simulink model "rate_channel"  (Simulink 4.00)
settings: Solver=ode45  StartTime=0.0  StopTime=100  RelTol=1e-3
libraries: simulink3 x2
settings Model: Creator=mcar  LastModifiedBy=mcar  BlockReductionOpt=off

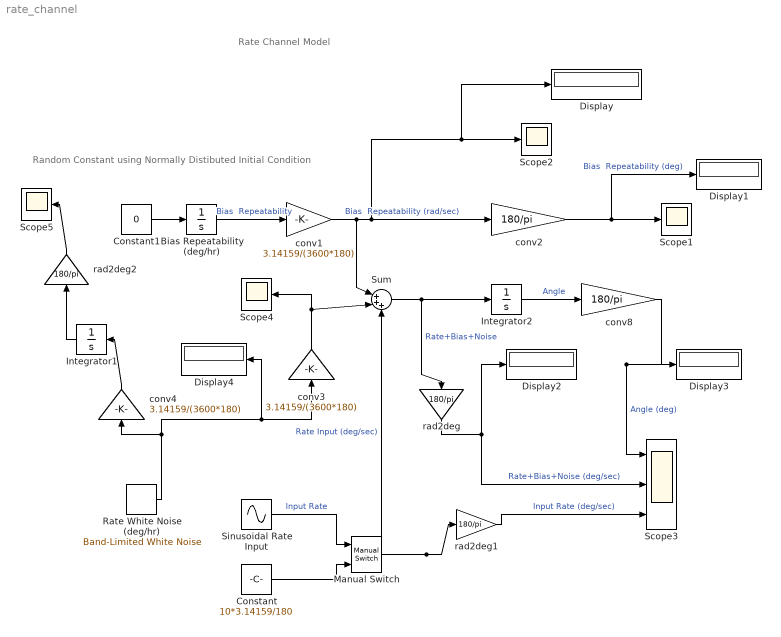
== system rate_channel ==
  note: Random Constant using
      | Normally Distibuted Initial Condition
  note: Rate Channel Model
  Bias Repeatability (deg/hr) : Integrator  ExternalReset=none  InitialConditionSource=internal  InitialCondition=10+3*rand  LimitOutput=off  UpperSaturationLimit=inf  LowerSaturationLimit=-inf  ShowSaturationPort=off  ShowStatePort=off  AbsoluteTolerance=auto
  Constant : Constant  Value=10*3.14159/180
  Constant1 : Constant  Value=0
  Display{,1..4} (5 alike) : Display
      settings: Format=short
  Integrator1 : Integrator  Orientation=left  ExternalReset=none  InitialConditionSource=internal  InitialCondition=0  LimitOutput=off  UpperSaturationLimit=inf  LowerSaturationLimit=-inf  ShowSaturationPort=off  ShowStatePort=off  AbsoluteTolerance=auto
  Integrator2 : Integrator  ExternalReset=none  InitialConditionSource=internal  InitialCondition=0  LimitOutput=off  UpperSaturationLimit=inf  LowerSaturationLimit=-inf  ShowSaturationPort=off  ShowStatePort=off  AbsoluteTolerance=auto
  Manual Switch : simulink3/Nonlinear/Manual Switch  sw=1  action=0
  Rate White Noise (deg/hr) : simulink3/Sources/Band-Limited White Noise  Cov=[360^2]  Ts=0.1  seed=[23341]
  Scope{1..2,4..5} (4 alike) : Scope
      Scope1 settings: TimeRange=auto  YMin=-5  YMax=5  SaveToWorkspace=off  SaveName=ScopeData  LimitDataPoints=on  MaxDataPoints=5000
      Scope2 settings: TimeRange=auto  YMin=-5  YMax=5  SaveToWorkspace=off  LimitDataPoints=on  MaxDataPoints=5000
      Scope4 settings: TimeRange=100  YMin=-0.02  YMax=0.03  SaveToWorkspace=off  SaveName=ScopeData3  LimitDataPoints=on  MaxDataPoints=5000
      Scope5 settings: TimeRange=auto  YMin=-5  YMax=5  SaveToWorkspace=off  SaveName=ScopeData4  LimitDataPoints=on  MaxDataPoints=5000
  Scope3 : Scope  NumInputPorts=3
      settings: TimeRange=auto  YMin=-0.1~-100~-100  YMax=0.8~100~100  SaveToWorkspace=off  SaveName=ScopeData2  LimitDataPoints=on  MaxDataPoints=5000
  Sinusoidal Rate Input : Sin  Amplitude=1  Frequency=10*pi/180/3600  Phase=0  SampleTime=0
  Sum : Sum  Inputs=|+++  SaturateOnIntegerOverflow=on
  conv1 : Gain  Gain=3.14159/(3600*180)  Multiplication=Element-wise(K.*u)  SaturateOnIntegerOverflow=on
  conv2 : Gain  Gain=180/pi  Multiplication=Element-wise(K.*u)  SaturateOnIntegerOverflow=on
  conv3 : Gain  Orientation=up  Gain=3.14159/(3600*180)  Multiplication=Element-wise(K.*u)  SaturateOnIntegerOverflow=on
  conv4 : Gain  Orientation=up  Gain=3.14159/(3600*180)  Multiplication=Element-wise(K.*u)  SaturateOnIntegerOverflow=on
  conv8 : Gain  Gain=180/pi  Multiplication=Element-wise(K.*u)  SaturateOnIntegerOverflow=on
  rad2deg : Gain  Orientation=down  Gain=180/pi  Multiplication=Element-wise(K.*u)  SaturateOnIntegerOverflow=on
  rad2deg1 : Gain  Gain=180/pi  Multiplication=Element-wise(K.*u)  SaturateOnIntegerOverflow=on
  rad2deg2 : Gain  Orientation=up  Gain=180/pi  Multiplication=Element-wise(K.*u)  SaturateOnIntegerOverflow=on
  wires:
  Bias Repeatability (deg/hr)/1 -> conv1/1  "Bias  Repeatability"
  Sum/1 -> Integrator2/1, rad2deg/1  "Rate+Bias+Noise"
  Rate White Noise (deg/hr)/1 -> conv3/1, Display4/1, conv4/1
  Integrator2/1 -> conv8/1  "Angle"
  conv8/1 -> Scope3/1, Display3/1  "Angle (deg)"
  conv1/1 -> Sum/1, conv2/1, Scope2/1, Display/1  "Bias  Repeatability (rad/sec)"
  conv2/1 -> Scope1/1, Display1/1  "Bias  Repeatability (deg)"
  conv3/1 -> Sum/2, Scope4/1
  rad2deg/1 -> Scope3/2, Display2/1  "Rate+Bias+Noise (deg/sec)"
  rad2deg1/1 -> Scope3/3  "Input Rate (deg/sec)"
  Constant/1 -> Manual Switch/2
  Sinusoidal Rate Input/1 -> Manual Switch/1  "Input Rate"
  Manual Switch/1 -> rad2deg1/1, Sum/3  "Rate Input (deg/sec)"
  Integrator1/1 -> rad2deg2/1
  conv4/1 -> Integrator1/1
  rad2deg2/1 -> Scope5/1
  Constant1/1 -> Bias Repeatability (deg/hr)/1
